simulink model "SIMmaboost"  (R2023b)
settings: Solver=VariableStepAuto  StartTime=0.0  StopTime=0.2  RelTol=1e-3
values from neighbouring files (symbols this model uses):
  C = 6.25e-05    [SimMAbosst.m]
  fs = 20000    [SimMAbosst.m]
  k = 50    [SimMAbosst.m]
  Vs = 30    [SimMAbosst.m]
libraries: spsSeriesRLCBranchLib x3, spsCurrentMeasurementLib x1, spsDiodeLib x1, spsDCVoltageSourceLib x1, spsGroundLib x1, spsMosfetLib x1, spsVoltageMeasurementLib x1, spspowerguiLib x1
settings Model: Creator=luisf  LastModifiedBy=luisf

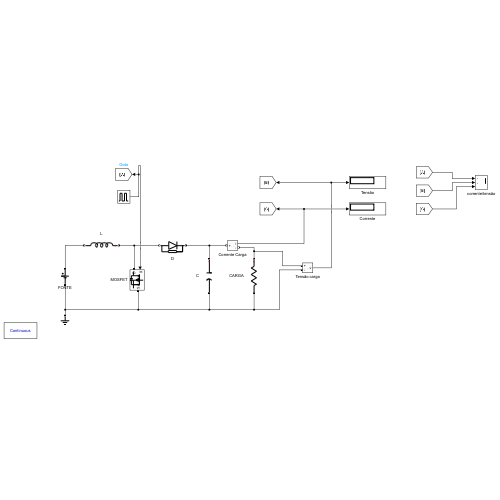
[thumbnail: Simulink's stored preview of the top-level diagram]
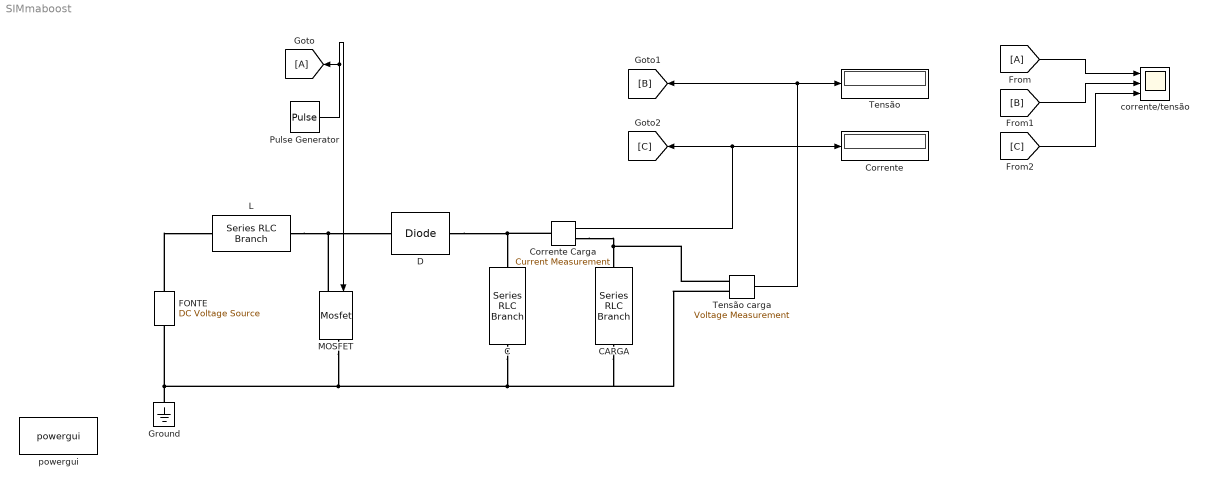
== system SIMmaboost ==
  C : spsSeriesRLCBranchLib/Series RLC Branch  LConnTagsString=__new0  RConnTagsString=__new0  BranchType=C  Resistance=1  Inductance=1e-3  SetiL0=off  InitialCurrent=0  Capacitance=C  Setx0=off  InitialVoltage=0  Measurements=None
  CARGA : spsSeriesRLCBranchLib/Series RLC Branch  LConnTagsString=__new0  RConnTagsString=__new0  BranchType=R  Resistance=15  Inductance=1e-3  SetiL0=off  InitialCurrent=0  Capacitance=1e-6  Setx0=off  InitialVoltage=0  Measurements=None
  Corrente : Display
  Corrente Carga : spsCurrentMeasurementLib/Current Measurement  PhasorSimulation=off  OutputType=Complex  PSBequivalent=0
  D : spsDiodeLib/Diode  Ron=0.001  Lon=0  Vf=1.7  IC=0  UseSnubber=0  Rs=500  Cs=250e-9  Measurements=off
  FONTE : spsDCVoltageSourceLib/DC Voltage Source  Amplitude=Vs  Measurements=None
  From : From
  Goto : Goto
  Ground : spsGroundLib/Ground  LConnTagsString=a
  L : spsSeriesRLCBranchLib/Series RLC Branch  LConnTagsString=__new0  RConnTagsString=__new0  BranchType=L  Resistance=1  Inductance=0.00056  SetiL0=off  InitialCurrent=0  Capacitance=1e-6  Setx0=off  InitialVoltage=0  Measurements=None
  MOSFET : spsMosfetLib/Mosfet  Ron=0.1  Lon=0  Rd=0.01  Vfd=0  IC=0  Rs=1e5  Cs=inf  Measurements=off
  Pulse Generator : DiscretePulseGenerator  PulseType=Time based  Period=1/fs  PulseWidth=k
  Tensão : Display
  Tensão carga : spsVoltageMeasurementLib/Voltage Measurement  PhasorSimulation=off  OutputType=Complex  PSBequivalent=0
  corrente/tensão : Scope  NumInputPorts=3
  powergui : spspowerguiLib/powergui  Priority=1  SimulationMode=Continuous  SampleTime=50e-6  frequency=60  Iterations=50  frequencyindice=0  Pbase=100e6  ErrMax=1e-4  UnitsV=kV  UnitsW=MW  buscounter=0  FunctionMessages=off  echomessages=off  EnableUseOfTLC=off  CurrentSourceSwitches=off  DisableSnubberDevices=off  DisableRonSwitches=off  DisableVfSwitches=off  DisplayEquations=off  AutomaticDiscreteSolvers=off  SolverType=Tustin/Backward Euler (TBE)  Interpol=off  ExternalGateDelay=off  methode=off  Ts=100  x0status=blocks  SPID=on  SwTol=0  HookPort=off  NonlinearTolerance=1e-4  nMaxIteration=100  ContinueOnMaxIteration=off  RestoreLinks=warning  ResistiveCurrentMeasurement=off  Frange=[0:2:500]  Ylog=off  Xlog=on  ShowGrid=off  save=off  variable=ZData  structure=0  ZoomFFT=off  StartTime=0.0  cycles=1  DisplayStyle=1  fundamental=60  FreqAxis=off  MaxFrequency=1000  frequencyindicesteady=1  RmsSteady=1  display=off
  wires:
  Pulse Generator/1 -> MOSFET/1, Goto/1
  From/1 -> corrente/tensão/1
  [B] -> corrente/tensão/2
  [C] -> corrente/tensão/3
  Tensão carga/1 -> Tensão/1, [B]
  Corrente Carga/1 -> [C], Corrente/1
  connections:
  Ground/LConn1 -- MOSFET/RConn1 -- Tensão carga/LConn2 -- CARGA/RConn1 -- C/RConn1 -- FONTE/LConn1
  FONTE/RConn1 -- L/RConn1
  L/LConn1 -- MOSFET/LConn1 -- D/LConn1
  D/RConn1 -- Corrente Carga/LConn1 -- C/LConn1
  Corrente Carga/RConn1 -- Tensão carga/LConn1 -- CARGA/LConn1
